simulink model "tip_assist_lib_support_angle_latch_concepting"  (Simulink 9.0)
settings: Solver=FixedStepDiscrete  StartTime=0.0  StopTime=10.0  FixedStep=.02  RelTol=1e-3
libraries: lib_CATutils_Hysteresis_Latch x1, tip_assist_lib_support x1
settings Model: Creator=CurriSD  LastModifiedBy=CurriSD
settings DataIOCC: SaveFormat=Dataset
settings OptimizationCC: LifeSpan=auto
settings DebuggingCC: UnderspecifiedInitializationDetection=Simplified  MergeDetectMultiDrivingBlocksExec=error  SFUnexpectedBacktrackingDiag=error  SFNoUnconditionalDefaultTransitionDiag=error  SFExecutionAtInitializationDiag=warning
settings HardwareCC: ProdBitPerPointer=64  ProdBitPerSizeT=64  ProdBitPerPtrDiffT=64  ProdLargestAtomicFloat=Float  ProdIntDivRoundTo=Zero  ProdEndianess=LittleEndian  ProdWordSize=64  ProdHWDeviceType=Intel->x86-64 (Windows64)
settings ModelReferenceCC: PropagateSignalLabelsOutOfModel=on
settings CodeAppCC: StateflowObjectComments=off
settings GRTTargetCC: TargetLangStandard=C99 (ISO)
settings ConfigComp: CovMetricSettings=dwe  CovHtmlReporting=off  CovSaveCumulativeToWorkspaceVar=off  CovSaveSingleToWorkspaceVar=off  CovExternalEMLEnable=on

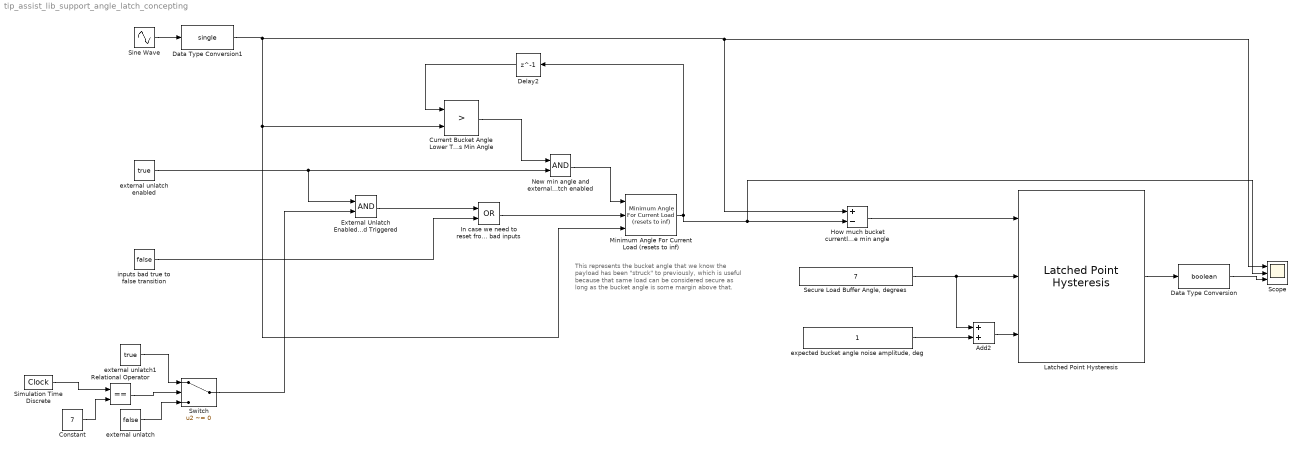
== system tip_assist_lib_support_angle_latch_concepting ==
  note: This represents the bucket angle that we know the payload has been "struck" to previously, which is useful because that same load can be considered secure as long as the bucket angle is some margin above that.
  Add2 : Sum
  Constant : Constant  Value=7
  Current Bucket Angle Lower Than Or Equal To Previous Min Angle : RelationalOperator  Operator=>  RndMeth=Nearest  InputSameDT=on
  Data Type Conversion : DataTypeConversion  OutDataTypeStr=boolean
  Data Type Conversion1 : DataTypeConversion  OutDataTypeStr=single
  Delay2 : Delay  DelayLength=1
  External Unlatch Enabled and Triggered : Logic  AllPortsSameDT=off  OutDataTypeStr=boolean
  How much bucket currently is above min angle : Sum  Inputs=+-
  In case we need to reset from bad inputs : Logic  Operator=OR  AllPortsSameDT=off  OutDataTypeStr=boolean
  Latched Point Hysteresis : lib_CATutils_Hysteresis_Latch/Latched Point Hysteresis  extBreakPoints=on  Min_Break_Point=-0.5  Max_Break_Point=0.5  extValues=off  Lo_Value=0  Hi_Value=1  Out_Mode=unused and invalid  Out_DataType=[]  Out_Scaling=[]  OutDataTypeStr=int8
  Minimum Angle For Current Load (resets to inf) : tip_assist_lib_support/Tip-Off Assist Support Lib/Tip-Off Assist Payload/Pseudo-Frictionless Weigh/Minimum Angle For Current Load (resets to inf)  mskInitialOut=single(inf)
  New min angle and external unlatch enabled : Logic  AllPortsSameDT=off  OutDataTypeStr=boolean
  Relational Operator : RelationalOperator  Operator===  OutDataTypeStr=boolean  RndMeth=Simplest
  Scope : Scope  NumInputPorts=3
  "Secure Load Buffer Angle, degrees" : Constant  Value=7  OutDataTypeStr=single  SampleTime=-1
  Simulation Time Discrete : DigitalClock  SampleTime=0.02
  Sine Wave : Sin  Amplitude=20  SampleTime=0
  Switch : Switch  Criteria=u2 ~= 0
  "expected bucket angle noise amplitude, deg" : Constant  OutDataTypeStr=single  SampleTime=-1
  external unlatch : Constant  Value=false
  external unlatch enabled : Constant  Value=true
  external unlatch1 : Constant  Value=true
  inputs bad true to false transition : Constant  Value=false
  wires:
  In case we need to reset from bad inputs/1 -> Minimum Angle For Current Load (resets to inf)/2
  External Unlatch Enabled and Triggered/1 -> In case we need to reset from bad inputs/1
  Add2/1 -> Latched Point Hysteresis/3
  "expected bucket angle noise amplitude, deg"/1 -> Add2/2
  How much bucket currently is above min angle/1 -> Latched Point Hysteresis/1
  Latched Point Hysteresis/1 -> Data Type Conversion/1
  Switch/1 -> External Unlatch Enabled and Triggered/2
  New min angle and external unlatch enabled/1 -> Minimum Angle For Current Load (resets to inf)/1
  inputs bad true to false transition/1 -> In case we need to reset from bad inputs/2
  Current Bucket Angle Lower Than Or Equal To Previous Min Angle/1 -> New min angle and external unlatch enabled/1
  external unlatch enabled/1 -> External Unlatch Enabled and Triggered/1, New min angle and external unlatch enabled/2
  "Secure Load Buffer Angle, degrees"/1 -> Latched Point Hysteresis/2, Add2/1
  Delay2/1 -> Current Bucket Angle Lower Than Or Equal To Previous Min Angle/1
  Sine Wave/1 -> Data Type Conversion1/1
  Minimum Angle For Current Load (resets to inf)/1 -> Scope/2, How much bucket currently is above min angle/2, Delay2/1
  Data Type Conversion/1 -> Scope/3
  Data Type Conversion1/1 -> Current Bucket Angle Lower Than Or Equal To Previous Min Angle/2, Minimum Angle For Current Load (resets to inf)/3, Scope/1, How much bucket currently is above min angle/1
  Simulation Time Discrete/1 -> Relational Operator/1
  Constant/1 -> Relational Operator/2
  Relational Operator/1 -> Switch/2
  external unlatch/1 -> Switch/3
  external unlatch1/1 -> Switch/1
